simulink model "ETA"  (R2024b)
settings: Solver=ode15s  StartTime=0.0  StopTime=1  MaxStep=0.01  RelTol=1e-3  AbsTol=1e-3  EnableMultiTasking=on
values from neighbouring files (symbols this model uses):
  m = [227.7, 160.8, 155.0, 152.0, 138.9, 130.6, 123.3, 114.7,        99.5,  93.2,  84.7,  75.5,  67.4,  59.2,  45.0,  38.6]    [print_properties.m]
  X = R .* cos(PHI + theta) + x    [single_tube_deflection.m]
  Y = R .* sin(PHI + theta)    [single_tube_deflection.m]
  Z = ones(size(X)) * z    [single_tube_deflection.m]
libraries: sm_lib x7, nesl_utility x2
settings Model: Creator=brice  LastModifiedBy=brice
settings SolverCC: AutoScaleAbsTol=off  AlgebraicLoopSolver=TrustRegion  MaxZcPerStep=1
settings DataIOCC: LimitDataPoints=on  MaxDataPoints=10000  TimeSaveName=t  OutputSaveName=y
settings OptimizationCC: ReuseModelBlockBuffer=off  LifeSpan=inf
settings DebuggingCC: AlgebraicLoopMsg=none  UnconnectedInputMsg=warning  UnconnectedOutputMsg=warning  UnconnectedLineMsg=warning  UniqueDataStoreMsg=error  AllowSymbolicDim=off  SubsystemReferenceDiagnosticForUnitTest=warning  SFUnexpectedBacktrackingDiag=warning  SFNoUnconditionalDefaultTransitionDiag=warning  SFExecutionAtInitializationDiag=none  ArithmeticOperatorsInVariantConditions=warning
settings ModelReferenceCC: EnableRefExpFcnMdlSchedulingChecks=on
settings SFSimCC: SimUseLocalCustomCode=off  CustomCodeUndefinedFunction=UseInterfaceOnly  SimTargetLang=C++
settings RTWCC: RTWUseLocalCustomCode=off  GPUComputeCapability=3.5  DLArmComputeVersion=19.05
settings CodeAppCC: StateflowObjectComments=on
settings GRTTargetCC: TargetLangStandard=C89/C90 (ANSI)
settings ConfigComp: CovMetricSettings=dw  CovSaveCumulativeToWorkspaceVar=on  CovSaveSingleToWorkspaceVar=on  CovExternalEMLEnable=off  CovSFcnEnable=off
settings SimscapeCC: SimscapeLogType=all  SimscapeLogSimulationStatistics=on  SimscapeLogDataHistory=10000
settings ExplorerConfigSet: InternalSimMechanicsExplorerSettings="<ExplorerConfiguration><canonicalview>planar_xy</canonicalview><AnimationSetting><BasePlaybackSpeed>1.0</BasePlaybackSpeed><PlaybackSpeedFactor>1.0</PlaybackSpeedFactor></AnimationSetting><TilePanel><TileInfo><Tiles Columns=\"1\" Count=\"1\" Rows=\"1\"><Column Weight=\"1\"/><Row Weight=\"1\"/><Tile Height=\"1\" Width=\"1\" X=\"0\" Y=\"0\"/></Tiles></TileInfo><SceneInfo><SceneViewer><BGColor><R>0.60000002384185791</R><G>0.60000002384185791</G><B>0.60000002384185791</B></BGColor><Camera><DoPerspective>off</DoPerspective><Position><X>-0.999999989712180071</X><Y>-0.0321560972250421809</Y><Z>0.439726779733458195</Z></Position><Center><X>1.02878198737776927e-08</X><Y>-0.0321560972250421809</Y><Z>0.439726779733458195</Z></Center><Up><X>-0</X><Y>1</Y><Z>0</Z></Up><ViewLimDist>1</ViewLimDist><YLim>0.361343014848777455</YLim><XLim>0.549485900399738658</XLim></Camera></SceneViewer></SceneInfo></TilePanel><MechEditorPanel><Cameras/><GfxPanelCameraMap/><VideoCreator><PlaybackSpeedRatio>1.0</PlaybackSpeedRatio><FrameRate>30</FrameRate><VideoFormat>Motion JPEG AVI</VideoFormat><FrameSize>auto</FrameSize></VideoCreator></MechEditorPanel></ExplorerConfiguration>"

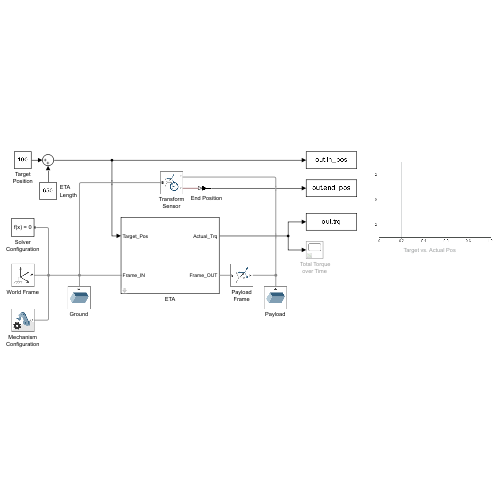
[thumbnail: Simulink's stored preview of the top-level diagram]
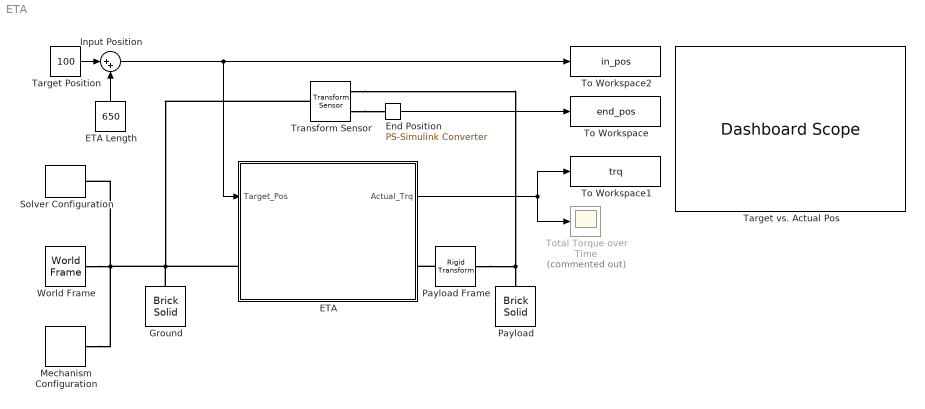
== system ETA ==
  " Total Torque over Time" : Scope  Commented=on
  ETA : Subsystem  mask{d_o=[13.4, 16.0, 18.3, 20.8, 23.3, 25.6, 28.3, 30.6, 33.2, 35.8, 38.3, 40.9, 43.6, 46.1, 48.9, 52.7], d_i=[12.2, 15.0, 17.0, 19.5, 22.0, 24.6, 27.0, 29.5, 32.0, 34.5, 37.0, 39.5, 42.3, 44.5, 47.5, 50.1], L=[600, 600, 640, 640, 640, 640, 640, 640, 640, 640, 640, 640, 640, 640, 640, 650], m=[38.6, 45.0, 59.2, 67.4, 75.5, 84.7, 93.2, 99.5, 114.7, 123.3, 130.6, 138.9, 152.0, 155.0, 160.8, 227.7], rho_gfrp=2370, E_gfrp=35.0, G_gfrp=5.0, rho_abs=1060, E_abs=2.0, G_abs=0.8}
      mask prompts: d_o "Outer Diameters (mm)"; d_i "Inner Diameters (mm)"; L "Lengths (mm)"; m "Weights (g)"; rho_gfrp "Density (kg/m^3)"; E_gfrp "Young's Modulus (GPa)"; G_gfrp "Shear Modulus (GPa)"; rho_abs "Density (kg/m^3)"; E_abs "Young's Modulus (GPa)"; G_abs "Shear Modulus (GPa)"
      mask DialogControl ParameterGroupVar Prompt: Physical Properties
      mask DialogControl ParameterSubgroup1Var Prompt: Mechanical Properties, GFRP (u_1-15)
      mask DialogControl ParameterSubgroup2Var Prompt: Mechanical Properties, ABS (u_16)
  ETA Length : Constant  Value=650
  End Position : nesl_utility/PS-Simulink Converter  PhysicalDomain=network_engine_domain  SubClassName=ps_output  LeftPortType=input  RightPortType=output  PseudoPeriodic=off  Frequencies=[]  VectorFormat=1-D array  Unit=mm  AffineConversion=off
  Ground : sm_lib/Body Elements/Brick Solid  BrickDimensions=[60 60 10]  BrickDimensionsUnits=mm  ExportEntireGeometry=off  InertiaType=CalculateFromGeometry  BasedOnType=Density  Density=1000  DensityUnits=kg/m^3  Mass=1  MassUnits=kg  CenterOfMass=[0 0 0]  CenterOfMassUnits=m  MomentsOfInertia=[1 1 1]  MomentsOfInertiaUnits=kg*m^2  ProductsOfInertia=[0 0 0]  ProductsOfInertiaUnits=kg*m^2  GraphicType=FromGeometry  MarkerShape=Sphere  MarkerSize=10  GraphicVisPropType=SimpleVisualProperties  GraphicDiffuseColor=[0.80 0.45 0]  GraphicOpacity=1.0  GraphicSpecularColor=[0.5 0.5 0.5 1.0]  GraphicAmbientColor=[0.15 0.15 0.15 1.0]  GraphicEmissiveColor=[0.0 0.0 0.0 1.0]  GraphicShininess=75  DoExposeReferenceFrame=on  SerializedFrames=<Frames/>
  Input Position : Sum  Inputs=|++
  Mechanism Configuration : sm_lib/Utilities/Mechanism Configuration  UniformGravity=Constant  GravityVector=[0 -9.80665 0]  GravityVectorUnits=m/s^2  LinearizationDelta=0.001  JointModeTransitionNonlinearIterations=2
  Payload : sm_lib/Body Elements/Brick Solid  BrickDimensions=[20 20 20]  BrickDimensionsUnits=mm  ExportEntireGeometry=off  InertiaType=PointMass  BasedOnType=Density  Density=1000  DensityUnits=kg/m^3  Mass=10000  MassUnits=g  CenterOfMass=[0 0 0]  CenterOfMassUnits=m  MomentsOfInertia=[1 1 1]  MomentsOfInertiaUnits=kg*m^2  ProductsOfInertia=[0 0 0]  ProductsOfInertiaUnits=kg*m^2  GraphicType=FromGeometry  MarkerShape=Sphere  MarkerSize=10  GraphicVisPropType=SimpleVisualProperties  GraphicDiffuseColor=[0 0.4471 0.7412]  GraphicOpacity=1.0  GraphicSpecularColor=[0.5 0.5 0.5 1.0]  GraphicAmbientColor=[0.15 0.15 0.15 1.0]  GraphicEmissiveColor=[0.0 0.0 0.0 1.0]  GraphicShininess=75  DoExposeReferenceFrame=on  SerializedFrames=<Frames/>
  Payload Frame : sm_lib/Frames and Transforms/Rigid Transform  RotationMethod=None  FollAlignAxisA=+X  BaseAlignAxisA=+Y  FollAlignAxisB=+Y  BaseAlignAxisB=+Z  RotationStandardAxis=+Z  RotationAngle=0.0  RotationAngleUnits=deg  RotationArbitraryAxis=[0 0 1]  RotationSequenceAxes=FollowerAxes  RotationSequence=XYX  RotationSequenceAngles=[0 0 0]  RotationSequenceAnglesUnits=deg  RotationMatrix=[1 0 0; 0 1 0; 0 0 1]  Quaternion=[1 0 0 0]  TranslationMethod=StandardAxis  TranslationCartesianOffset=[0 0 0]  TranslationCartesianOffsetUnits=m  TranslationStandardAxis=+Z  TranslationStandardOffset=600 + 10  TranslationStandardOffsetUnits=mm  TranslationROffset=0  TranslationROffsetUnits=m  TranslationThetaOffset=0  TranslationThetaOffsetUnits=deg  TranslationZOffset=0  TranslationZOffsetUnits=m
  Solver Configuration : nesl_utility/Solver Configuration  PhysicalDomain=network_engine_domain  SubClassName=solver  LeftPortType=input  RightPortType=generic  Tones=[]  Harmonics=[]  SimulateNoise=off  Profile=off  UseLocalSampling=off  EnableSwitchedLinearOptims=on  FrequencyDomain=off  UseCCode=off  RelTol=0.001  AbsTol=1e-06  MinStep=1e-09  ToWorkspace=off  RevertToSquareIcSolve=off  NumHomotopyIterations=100  PhasorMode=off  PhasorModeNumHarmonics=1  ConsistencySolver=NEWTON_XTOL_AFTER_FTOL  IndexReductionMethod=DerivativeReplacement  DoDC=off  ResidualTolerance=1e-09  ConsistencyTolSource=GLOBAL  ConsistencyAbsTol=0.001  ConsistencyRelTol=0.001  ConsistencyTolFactor=0.001  UseLocalSolver=off  LocalSolverChoice=NE_BACKWARD_EULER_ADVANCER  ResolveIndetEquations=on  FunctionEvalNumThread=1  LocalSolverSampleTime=0.001  DoFixedCost=off  MaxNonlinIter=3  MaxModeIter=2  ComputeImpulses=off  ImpulseIterations=2  LinearAlgebra=auto  LinearAlgebraNumThread=0  EquationFormulation=NE_TIME_EF  DelaysMemoryBudget=1024  AutomaticFiltering=on  FilteringTimeConstant=0.001  PartitionStorageMethod=AS_NEEDED  PartitionMemoryBudget=1024  PartitionMethod=FAST  MultibodyUseLocalSolver=off  MultibodyLocalSolverChoice=ODE1  MultibodyLocalSolverSampleTime=0.001
  Target Position : Constant  Value=100
  Target vs. Actual Pos : DashboardScope  UpdateMode=Scroll  NormalizeYAxis=on  Markers=on
  To Workspace : ToWorkspace  VariableName=end_pos  SaveFormat=Timeseries  SampleTime=-1
  To Workspace1 : ToWorkspace  VariableName=trq  SaveFormat=Timeseries  SampleTime=-1
  To Workspace2 : ToWorkspace  VariableName=in_pos  SaveFormat=Timeseries  SampleTime=-1
  Transform Sensor : sm_lib/Frames and Transforms/Transform Sensor  MeasurementFrame=World  RotationSequence=XYX  SenseAngle=off  SenseAxis=off  SenseQ=off  SenseR=off  SenseRotationSequence=off  SenseOmegaX=off  SenseOmegaY=off  SenseOmegaZ=off  SenseOmega=off  SenseQDot=off  SenseRDot=off  SenseRotationSequenceDot=off  SenseAlphaX=off  SenseAlphaY=off  SenseAlphaZ=off  SenseAlpha=off  SenseQDDot=off  SenseRDDot=off  SenseX=off  SenseY=off  SenseZ=on  SenseXYZ=off  SenseRad=off  SenseAzim=off  SenseDist=off  SenseInc=off  SenseXDot=off  SenseYDot=off  SenseZDot=off  SenseXYZDot=off  SenseRadDot=off  SenseAzimDot=off  SenseDistDot=off  SenseIncDot=off  SenseXDDot=off  SenseYDDot=off  SenseZDDot=off  SenseXYZDDot=off  SenseRadDDot=off  SenseAzimDDot=off  SenseDistDDot=off  SenseIncDDot=off
  World Frame : sm_lib/Frames and Transforms/World Frame
  wires:
  Input Position/1 -> ETA/1(Target_Pos), To Workspace2/1
  ETA/1(Actual_Trq) -> " Total Torque over Time"/1, To Workspace1/1
  End Position/1 -> To Workspace/1
  Target Position/1 -> Input Position/1
  ETA Length/1 -> Input Position/2
  connections:
  Transform Sensor/RConn2 -- End Position/LConn1
  Transform Sensor/LConn1 -- ETA/LConn1 -- Ground/RConn1 -- World Frame/RConn1 -- Mechanism Configuration/RConn1 -- Solver Configuration/RConn1
  Transform Sensor/RConn1 -- Payload Frame/RConn1 -- Payload/RConn1
  Payload Frame/LConn1 -- ETA/RConn1

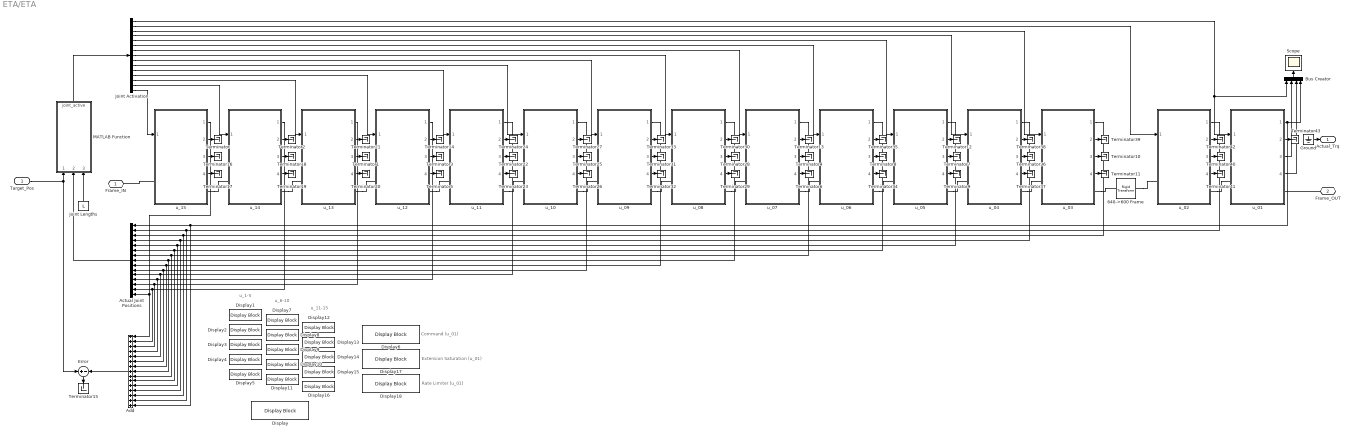
== system ETA/ETA ==
  note: u_1-5
  note: u_6-10
  note: u_11-15
  note: Command (u_01)
  note: Extension Saturation (u_01)
  note: Rate Limiter (u_01)
  Target_Pos : Inport
  640->600 Frame : sm_lib/Frames and Transforms/Rigid Transform  RotationMethod=None  FollAlignAxisA=+X  BaseAlignAxisA=+Y  FollAlignAxisB=+Y  BaseAlignAxisB=+Z  RotationStandardAxis=+Z  RotationAngle=0.0  RotationAngleUnits=deg  RotationArbitraryAxis=[0 0 1]  RotationSequenceAxes=FollowerAxes  RotationSequence=XYX  RotationSequenceAngles=[0 0 0]  RotationSequenceAnglesUnits=deg  RotationMatrix=[1 0 0; 0 1 0; 0 0 1]  Quaternion=[1 0 0 0]  TranslationMethod=StandardAxis  TranslationCartesianOffset=[0 0 0]  TranslationCartesianOffsetUnits=m  TranslationStandardAxis=+Z  TranslationStandardOffset=40  TranslationStandardOffsetUnits=mm  TranslationROffset=0  TranslationROffsetUnits=m  TranslationThetaOffset=0  TranslationThetaOffsetUnits=deg  TranslationZOffset=0  TranslationZOffsetUnits=m
  Actual Joint Positions : Mux  Inputs=15
  Add : Sum  Inputs=+++++++++++++++
  Bus Creator : BusCreator  Inputs=4
  Display : DisplayBlock  LabelPosition=Bottom  Format=Custom  Transparency=1  FormatString=%0.3f
  Display{1..5,7..16} (15 alike) : DisplayBlock  LabelPosition=Hide  Format=Custom  Transparency=1  FormatString=%0.1f
  Display17 : DisplayBlock  LabelPosition=Hide  Format=Custom  Transparency=1  FormatString=%0.3f
  Display18 : DisplayBlock  LabelPosition=Hide  Format=Custom  Transparency=1  FormatString=%0.3f
  Display6 : DisplayBlock  LabelPosition=Hide  Format=Custom  Transparency=1  FormatString=%0.3f
  Error : Sum  Inputs=+|-
  Ground : Ground
  Joint Activation : Demux  Outputs=15
  Joint Lengths : Constant  Value=L
  MATLAB Function : MATLAB Function  TreatAsAtomicUnit=on
  Scope : Scope
  Terminator{,1..43} (44 alike) : Terminator
  u_01 : Subsystem  ReferencedSubsystem=Telescoping_Tube  i=1
  u_02 : Subsystem  ReferencedSubsystem=Telescoping_Tube  i=2
  u_03 : Subsystem  ReferencedSubsystem=Telescoping_Tube  i=3
  u_04 : Subsystem  ReferencedSubsystem=Telescoping_Tube  i=4
  u_05 : Subsystem  ReferencedSubsystem=Telescoping_Tube  i=5
  u_06 : Subsystem  ReferencedSubsystem=Telescoping_Tube  i=6
  u_07 : Subsystem  ReferencedSubsystem=Telescoping_Tube  i=7
  u_08 : Subsystem  ReferencedSubsystem=Telescoping_Tube  i=8
  u_09 : Subsystem  ReferencedSubsystem=Telescoping_Tube  i=9
  u_10 : Subsystem  ReferencedSubsystem=Telescoping_Tube  i=10
  u_11 : Subsystem  ReferencedSubsystem=Telescoping_Tube  i=11
  u_12 : Subsystem  ReferencedSubsystem=Telescoping_Tube  i=12
  u_13 : Subsystem  ReferencedSubsystem=Telescoping_Tube  i=13
  u_14 : Subsystem  ReferencedSubsystem=Telescoping_Tube  i=14
  u_15 : Subsystem  ReferencedSubsystem=Telescoping_Tube  i=15
  Frame_IN : PMIOPort  Side=Left
  Frame_OUT : PMIOPort  Port=2  Side=Right
  Actual_Trq : Outport
  wires:
  Actual Joint Positions/1 -> MATLAB Function/2(actual_pos)
  MATLAB Function/1(joint_active) -> Joint Activation/1
  u_14/1 -> Add/2, Actual Joint Positions/14
  u_13/1 -> Actual Joint Positions/13, Add/3
  u_11/1 -> Actual Joint Positions/11, Add/5
  u_10/1 -> Actual Joint Positions/10, Add/6
  u_09/1 -> Actual Joint Positions/9, Add/7
  u_08/1 -> Actual Joint Positions/8, Add/8
  u_07/1 -> Actual Joint Positions/7, Add/9
  u_06/1 -> Add/10, Actual Joint Positions/6
  u_05/1 -> Add/11, Actual Joint Positions/5
  u_04/1 -> Add/12, Actual Joint Positions/4
  u_03/1 -> Add/13, Actual Joint Positions/3
  u_02/1 -> Add/14, Actual Joint Positions/2
  u_01/1 -> Bus Creator/4, Actual Joint Positions/1, Add/15
  Target_Pos/1 -> MATLAB Function/1(target_pos), Error/1
  u_12/1 -> Actual Joint Positions/12, Add/4
  Joint Lengths/1 -> MATLAB Function/3(joint_len)
  u_15/1 -> Add/1, Actual Joint Positions/15
  Add/1 -> Error/2
  Error/1 -> Terminator15/1
  Joint Activation/1 -> Bus Creator/1, u_01/1
  Joint Activation/13 -> u_13/1
  Joint Activation/11 -> u_11/1
  Joint Activation/7 -> u_07/1
  Joint Activation/9 -> u_09/1
  Joint Activation/8 -> u_08/1
  Joint Activation/6 -> u_06/1
  Joint Activation/5 -> u_05/1
  Joint Activation/15 -> u_15/1
  Joint Activation/14 -> u_14/1
  Joint Activation/12 -> u_12/1
  Joint Activation/10 -> u_10/1
  Joint Activation/3 -> u_03/1
  Joint Activation/4 -> u_04/1
  Joint Activation/2 -> u_02/1
  u_15/2 -> Terminator/1
  u_15/3 -> Terminator16/1
  u_15/4 -> Terminator17/1
  u_14/2 -> Terminator2/1
  u_14/3 -> Terminator18/1
  u_14/4 -> Terminator19/1
  u_13/3 -> Terminator1/1
  u_13/2 -> Terminator21/1
  u_13/4 -> Terminator20/1
  u_12/2 -> Terminator14/1
  u_12/3 -> Terminator3/1
  u_12/4 -> Terminator5/1
  u_11/2 -> Terminator24/1
  u_11/3 -> Terminator22/1
  u_11/4 -> Terminator23/1
  u_10/3 -> Terminator25/1
  u_10/2 -> Terminator27/1
  u_10/4 -> Terminator26/1
  u_07/3 -> Terminator4/1
  u_07/2 -> Terminator13/1
  u_07/4 -> Terminator6/1
  u_08/2 -> Terminator30/1
  u_08/3 -> Terminator28/1
  u_08/4 -> Terminator29/1
  u_09/2 -> Terminator33/1
  u_09/3 -> Terminator31/1
  u_09/4 -> Terminator32/1
  u_06/3 -> Terminator8/1
  u_06/2 -> Terminator35/1
  u_06/4 -> Terminator34/1
  u_05/3 -> Terminator7/1
  u_05/2 -> Terminator12/1
  u_05/4 -> Terminator9/1
  u_04/3 -> Terminator36/1
  u_04/2 -> Terminator38/1
  u_04/4 -> Terminator37/1
  u_03/2 -> Terminator39/1
  u_03/3 -> Terminator10/1
  u_03/4 -> Terminator11/1
  u_02/3 -> Terminator40/1
  u_02/2 -> Terminator42/1
  u_02/4 -> Terminator41/1
  u_01/2 -> Terminator43/1
  u_01/4 -> Bus Creator/3
  u_01/3 -> Bus Creator/2
  Bus Creator/1 -> Scope/1
  Ground/1 -> Actual_Trq/1
  connections:
  u_15/LConn1 -- Frame_IN/RConn1
  u_15/RConn1 -- u_14/LConn1
  u_13/RConn1 -- u_12/LConn1
  u_14/RConn1 -- u_13/LConn1
  u_11/RConn1 -- u_10/LConn1
  u_10/RConn1 -- u_09/LConn1
  u_09/RConn1 -- u_08/LConn1
  u_12/RConn1 -- u_11/LConn1
  u_04/RConn1 -- u_03/LConn1
  u_02/RConn1 -- u_01/LConn1
  u_07/RConn1 -- u_06/LConn1
  u_06/RConn1 -- u_05/LConn1
  u_05/RConn1 -- u_04/LConn1
  u_08/RConn1 -- u_07/LConn1
  Frame_OUT/RConn1 -- u_01/RConn1
  u_03/RConn1 -- 640->600 Frame/LConn1
  640->600 Frame/RConn1 -- u_02/LConn1

== matlab function ETA/MATLAB Function ==
  data: target_pos input; joint_active output; actual_pos input; joint_len input
% ETA Control Logic
%   @param target_pos Target length of the ETA, in mm (scalar)
%   @param actual_pos Current joint positions, in mm (1D array)
%   @param joint_len Joint lengths, in mm (1D array)
%   @return joint_active Commanded joint, '1' for enabled/'0' for disabled (1-D array)
%
function joint_active = controlLogic(target_pos, actual_pos, joint_len)
    % Initialize local variables
    error = target_pos - sum(actual_pos);  % difference btw. target and actual
    N = length(actual_pos);  % number of joints
    joint_max = joint_len - 150;  % max extension for each joint, in mm

    joint_active = zeros(N, 1);
    
    if error > 0
        for i = 1:N  % extend, smallest first
            if actual_pos(i) < joint_max(i)
                joint_active(i) = joint_max(i);
                break;  % only one joint should move at a time
            end
        end
    elseif error < 0
        for i = N:-1:1  % retract, largest first
            if actual_pos(i) > 0
                if actual_pos(i) > 0
                    joint_active(i) = 0;
                    break;  % only one joint should move at a time
                end
            end
        end
    end
end
